simulink model "BEV_Milg_OctNov24"  (R2024b)
settings: Solver=ode23tb  StartTime=0.0  StopTime=100000  RelTol=1e-3
InitFcn:
  | P=200;
  | i_g=11;
  | Battery_C=53;
  | 
  | m=2208;
  | c=.29;
  | frr=0.02;
  | g=9.81;
  | Cmax=Battery_C*1e3/340;
  | et=0.9;
  | rw=.37;
libraries: simulink x1, autolibshared x1, slpidlib x1
settings Model: Creator=Kamyar  LastModifiedBy=samar
settings SolverCC: AlgebraicLoopSolver=TrustRegion
settings DebuggingCC: UnconnectedInputMsg=warning  UnconnectedOutputMsg=warning  UnconnectedLineMsg=warning
settings ModelReferenceCC: EnableRefExpFcnMdlSchedulingChecks=on
settings RTWCC: GPUComputeCapability=3.5  DLArmComputeVersion=19.05

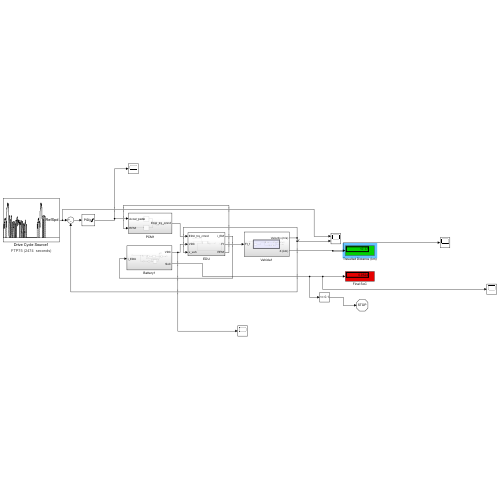
[thumbnail: Simulink's stored preview of the top-level diagram]
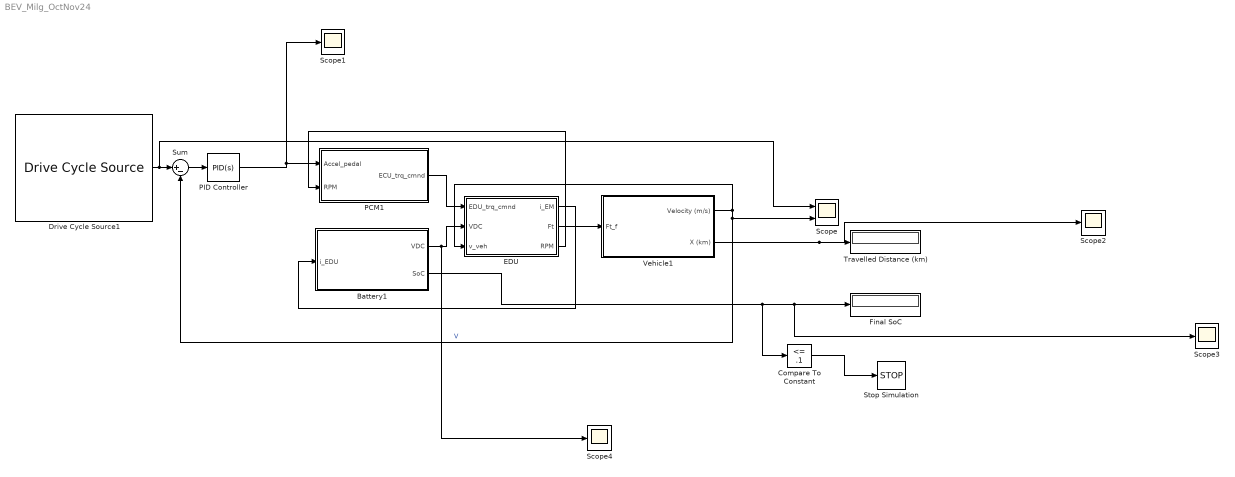
== system BEV_Milg_OctNov24 ==
  Battery1 : Subsystem
  Compare To Constant : simulink/Logic and Bit Operations/Compare To Constant  relop=<=  const=.1  OutDataTypeStr=boolean
  Drive Cycle Source1 : autolibshared/Drive Cycle Source  cycleVar=FTP75  fileVar=cycleFTP75.mat  tfinal="2474  seconds"  cycleRepeat=off  outAccPort=off  outGearPort=off  gearList=No gear data  t_wot1=5  xdot_woto=0  xdot_wot1=30  t_wot2=20  xdot_wot2=0  t_wotend=30  srcUnit=m/s  outUnit=m/s  srcAccUnit=m/s/s  outAccUnit=m/s^2  dt=0  aMode=1  faultOption=off  velBnd=2  velBndUnit=mph  inUnit=m/s  timeBnd=1  failOption=off  stopSim=off  maxFaultCnt=10  maxFaultTime=2  maxTotFaultTime=15  traceOption=off  dtTrace=1  traceWindow=10  lastDCname=FTP75  lastOutUnit=mph  lastDT=0  lastTB=1  lastSB=2  forceCalcBound=off
  EDU : Subsystem
  Final SoC : Display
  PCM1 : Subsystem
  PID Controller : slpidlib/PID Controller  Controller=PID  Form=Parallel  TimeDomain=Continuous-time  UseExternalTs=off  SampleTime=-1  IntegratorMethod=Forward Euler  FilterMethod=Forward Euler  ControllerParametersSource=internal  P=.1  I=.05  UseKiTs=off  D=0  UseExternalDerivativeSource=off  N=100  UseFilter=on  TunerSelectOption=Transfer Function Based (PID Tuner App)  InitialConditionSource=internal  InitialConditionForIntegrator=0  InitialConditionForFilter=0  DifferentiatorICPrevScaledInput=0  ExternalReset=none  TrackingMode=off  Kt=1  LimitOutput=on  SatLimitsSource=internal  UpperSaturationLimit=1  LowerSaturationLimit=-1  LinearizeAsGain=on  AntiWindupMode=back-calculation  Kb=2  LimitIntegrator=off  UpperIntegratorSaturationLimit=inf  LowerIntegratorSaturationLimit=-inf  POutMin=[]  POutMax=[]  IOutMin=[]  IOutMax=[]  DOutMin=[]  DOutMax=[]  NOutMin=[]  NOutMax=[]  SumOutMin=[]  SumOutMax=[]  SaturationOutMin=[]  SaturationOutMax=[]  PParamMin=[]  PParamMax=[]  IParamMin=[]  IParamMax=[]  DParamMin=[]  DParamMax=[]  NParamMin=[]  NParamMax=[]  KbParamMin=[]  KbParamMax=[]  KtParamMin=[]  KtParamMax=[]  KbOutMin=[]  KbOutMax=[]  KtOutMin=[]  KtOutMax=[]  IntegratorOutMin=[]  IntegratorOutMax=[]  FilterOutMin=[]  FilterOutMax=[]  SumI1OutMin=[]  SumI1OutMax=[]  SumI2OutMin=[]  SumI2OutMax=[]  SumI3OutMin=[]  SumI3OutMax=[]  SumI4OutMin=[]  SumI4OutMax=[]  SumDOutMin=[]  SumDOutMax=[]  DifferentiatorOutMin=[]  DifferentiatorOutMax=[]  FilterDiffOutCoefMin=[]  FilterDiffOutCoefMax=[]  ReciprocalOutMin=[]  ReciprocalOutMax=[]  SumDenOutMin=[]  SumDenOutMax=[]  SumNumOutMin=[]  SumNumOutMax=[]  DivideOutMin=[]  DivideOutMax=[]  UdiffTsProdOutMin=[]  UdiffTsProdOutMax=[]  NTsProdOutMin=[]  NTsProdOutMax=[]  UintegralTsProdOutMin=[]  UintegralTsProdOutMax=[]  UngainTsProdOutMin=[]  UngainTsProdOutMax=[]  ClampingZeroOutDataTypeStr=Inherit: Inherit via back propagation  ClampingZeroOutMin=[]  ClampingZeroOutMax=[]  FilterDenConstantOutDataTypeStr=Inherit: Inherit via back propagation  FilterDenConstantOutMin=[]  FilterDenConstantOutMax=[]  PCopyOutDataTypeStr=Inherit: Inherit via back propagation  PCopyOutMin=[]  PCopyOutMax=[]  NCopyOutDataTypeStr=Inherit: Inherit via back propagation  NCopyOutMin=[]  NCopyOutMax=[]  IntegratorContinuousStateAttributes=''  IntegratorStateMustResolveToSignalObject=off  IntegratorRTWStateStorageClass=Auto  FilterContinuousStateAttributes=''  FilterStateMustResolveToSignalObject=off  FilterRTWStateStorageClass=Auto  ParallelPVariant=InternalParameters  IdealPVariant=Disabled  IVariant=InternalParameters  DVariant=InternalParameters  IntegratorVariant=Continuous  SatVariant=Enabled  AWVariant=BackCalculation  PCopyVariant=Disabled  TRVariant=Disabled  FdbkBlocksVariant=Forward  IdealPFdbkVariant=Disabled  SatFdbkVariant=Disabled  DerivativeFilterVariant=ContFilter  NVariant=InternalParameters  NCopyVariant=Disabled  FilterICVariant=InternalICsFilter  IntegratorICVariant=InternalICs  ExternalResetVariant=Disabled  TRSumVariant=Passthrough  SumFdbkVariant=Disabled  SumVariant=Sum_PID  TsampFilterVariant=InternalTs  TsampNgainVariant=Passthrough  TsampIntegralVariant=Disabled_SignalSpec  ExternalSaturationOutDataTypeStr=Inherit: Same as second input  DerivativeSourceVariant=ErrorSignal  PreIntVariant=InternalPreInt
  Scope : Scope  NumInputPorts=2
  Scope{1..4} (4 alike) : Scope
  Stop Simulation : Stop
  Sum : Sum  Inputs=|+-
  Travelled Distance (km) : Display
  Vehicle1 : Subsystem
  wires:
  Sum/1 -> PID Controller/1
  Drive Cycle Source1/1 -> Scope/1, Sum/1
  Vehicle1/1(Velocity (m/s)) -> Scope/2, Sum/2, EDU/3(v_veh)  "V"
  PID Controller/1 -> PCM1/1(Accel_pedal), Scope1/1
  Vehicle1/2(X (km)) -> Scope2/1, Travelled Distance (km)/1
  PCM1/1(ECU_trq_cmnd) -> EDU/1(EDU_trq_cmnd)
  Battery1/1(VDC) -> Scope4/1, EDU/2(VDC)
  EDU/2(Ft) -> Vehicle1/1(Ft_f)
  EDU/1(i_EM) -> Battery1/1(i_EDU)
  EDU/3(RPM) -> PCM1/2(RPM)
  Compare To Constant/1 -> Stop Simulation/1
  Battery1/2(SoC) -> Compare To Constant/1, Scope3/1, Final SoC/1

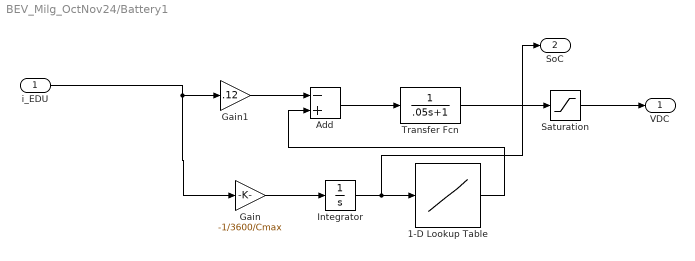
== system BEV_Milg_OctNov24/Battery1 ==
  i_EDU : Inport
  1-D Lookup Table : Lookup_n-D  NumberOfTableDimensions=1  BreakpointsForDimension1=|  Table=|  InternalRulePriority=Speed  RndMeth=Simplest
      BreakpointsForDimension1=|
      | [0
      | 0.028708134
      | 0.04784689
      | 0.105263158
      | 0.207336523
      | 0.398724083
      | 0.535885167
      | 0.596491228
      | 0.68261563
      | 0.797448166
      | 1
      | ]
      Table=|
      | [279.7468354
      | 298.9873418
      | 313.164557
      | 323.0379747
      | 330.6329114
      | 339.7468354
      | 344.556962
      | 347.8481013
      | 356.4556962
      | 367.0886076
      | 391.1392405
      | ]
  Add : Sum  Inputs=-+
  Gain : Gain  Gain=-1/3600/Cmax
  Gain1 : Gain  Gain=.12
  Integrator : Integrator  InitialCondition=1
  Saturation : Saturate  UpperLimit=inf  LowerLimit=200
  Transfer Fcn : TransferFcn  Denominator=[.05 1]
  VDC : Outport
  SoC : Outport  Port=2
  wires:
  i_EDU/1 -> Gain/1, Gain1/1
  Gain/1 -> Integrator/1
  Integrator/1 -> SoC/1, 1-D Lookup Table/1
  1-D Lookup Table/1 -> Add/2
  Gain1/1 -> Add/1
  Add/1 -> Transfer Fcn/1
  Transfer Fcn/1 -> Saturation/1
  Saturation/1 -> VDC/1

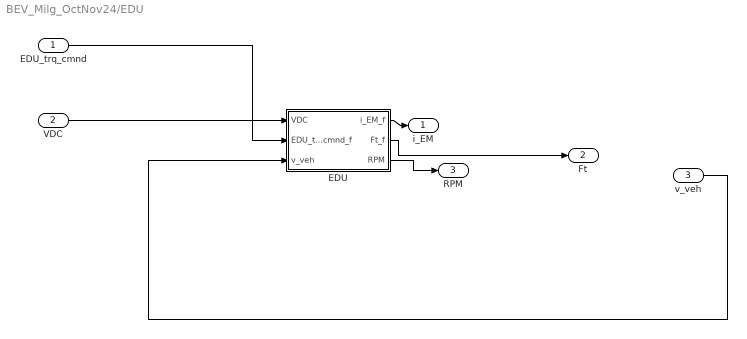
== system BEV_Milg_OctNov24/EDU ==
  EDU_trq_cmnd : Inport
  VDC : Inport  Port=2
  v_veh : Inport  Port=3
  " EDU" : Subsystem
  i_EM : Outport
  Ft : Outport  Port=2
  RPM : Outport  Port=3
  wires:
  " EDU"/2(Ft_f) -> Ft/1
  VDC/1 -> " EDU"/1(VDC)
  v_veh/1 -> " EDU"/3(v_veh)
  " EDU"/1(i_EM_f) -> i_EM/1
  EDU_trq_cmnd/1 -> " EDU"/2(EDU_trq_cmnd_f)
  " EDU"/3(RPM) -> RPM/1

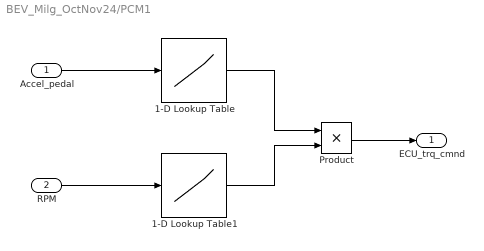
== system BEV_Milg_OctNov24/PCM1 ==
  Accel_pedal : Inport
  RPM : Inport  Port=2
  1-D Lookup Table : Lookup_n-D  NumberOfTableDimensions=1  BreakpointsForDimension1=0:.2:1  Table=[0 .4 .6 .825 .95 1]  InternalRulePriority=Speed  RndMeth=Simplest
  1-D Lookup Table1 : Lookup_n-D  NumberOfTableDimensions=1  BreakpointsForDimension1=[0:500:13000]  Table=[ones(1,9)*P*1e3/4000/(pi/30),P*1e3/(pi/30)./[4500:500:13000]]  InternalRulePriority=Speed  RndMeth=Simplest
  Product : Product
  ECU_trq_cmnd : Outport
  wires:
  Accel_pedal/1 -> 1-D Lookup Table/1
  1-D Lookup Table1/1 -> Product/2
  1-D Lookup Table/1 -> Product/1
  Product/1 -> ECU_trq_cmnd/1
  RPM/1 -> 1-D Lookup Table1/1

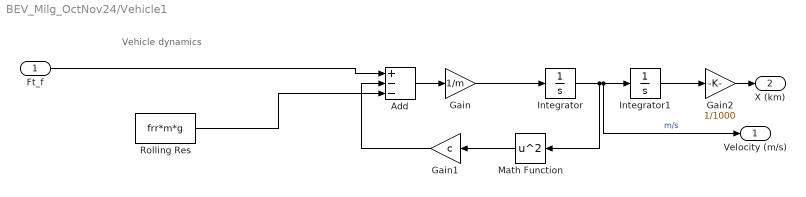
== system BEV_Milg_OctNov24/Vehicle1 ==
  note: Vehicle dynamics
  Ft_f : Inport
  Add : Sum  Inputs=+--
  Gain : Gain  Gain=1/m
  Gain1 : Gain  Gain=c
  Gain2 : Gain  Gain=1/1000
  Integrator : Integrator
  Integrator1 : Integrator
  Math Function : Math  Operator=square
  Rolling Res : Constant  Value=frr*m*g
  Velocity (m/s) : Outport
  X (km) : Outport  Port=2
  wires:
  Gain/1 -> Integrator/1
  Add/1 -> Gain/1
  Gain1/1 -> Add/2
  Integrator/1 -> Math Function/1, Velocity (m/s)/1, Integrator1/1  "m/s"
  Math Function/1 -> Gain1/1
  Ft_f/1 -> Add/1
  Gain2/1 -> X (km)/1
  Integrator1/1 -> Gain2/1
  Rolling Res/1 -> Add/3

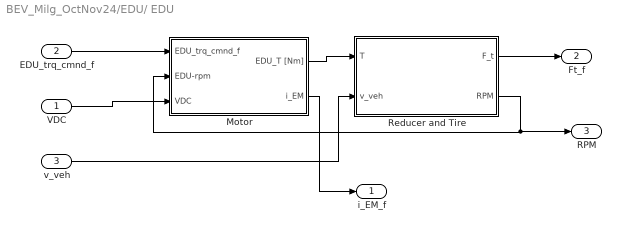
== system BEV_Milg_OctNov24/EDU/ EDU ==
  VDC : Inport
  EDU_trq_cmnd_f : Inport  Port=2
  v_veh : Inport  Port=3
  Motor : Subsystem
  Reducer and Tire : Subsystem
  i_EM_f : Outport
  Ft_f : Outport  Port=2
  RPM : Outport  Port=3
  wires:
  Motor/2(i_EM) -> i_EM_f/1
  Reducer and Tire/1(F_t) -> Ft_f/1
  Reducer and Tire/2(RPM) -> RPM/1, Motor/2(EDU-rpm)
  v_veh/1 -> Reducer and Tire/2(v_veh)
  Motor/1(EDU_T [Nm]) -> Reducer and Tire/1(T)
  VDC/1 -> Motor/3(VDC)
  EDU_trq_cmnd_f/1 -> Motor/1(EDU_trq_cmnd_f)

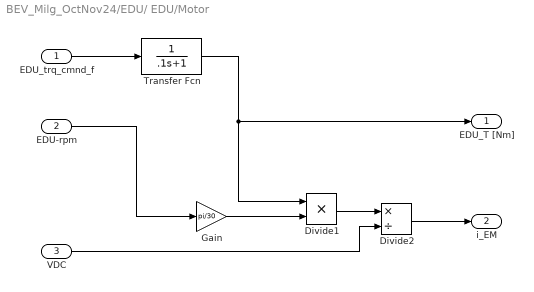
== system BEV_Milg_OctNov24/EDU/ EDU/Motor ==
  EDU_trq_cmnd_f : Inport
  EDU-rpm : Inport  Port=2
  VDC : Inport  Port=3
  Divide1 : Product
  Divide2 : Product  Inputs=*/
  Gain : Gain  Gain=pi/30
  Transfer Fcn : TransferFcn  Denominator=[.1 1]
  EDU_T [Nm] : Outport
  i_EM : Outport  Port=2
  wires:
  EDU-rpm/1 -> Gain/1
  EDU_trq_cmnd_f/1 -> Transfer Fcn/1
  Divide1/1 -> Divide2/1
  Divide2/1 -> i_EM/1
  VDC/1 -> Divide2/2
  Gain/1 -> Divide1/2
  Transfer Fcn/1 -> Divide1/1, EDU_T [Nm]/1

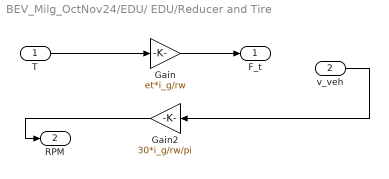
== system BEV_Milg_OctNov24/EDU/ EDU/Reducer and Tire ==
  T : Inport
  v_veh : Inport  Port=2
  Gain : Gain  Gain=et*i_g/rw
  Gain2 : Gain  Gain=30*i_g/rw/pi
  F_t : Outport
  RPM : Outport  Port=2
  wires:
  Gain2/1 -> RPM/1
  T/1 -> Gain/1
  v_veh/1 -> Gain2/1
  Gain/1 -> F_t/1
